simulink model "task3_lab7"  (R2024b)
settings: Solver=VariableStepAuto  StartTime=0.0  StopTime=10.0  RelTol=1e-3
settings Model: Creator=Beanie  LastModifiedBy=Beanie

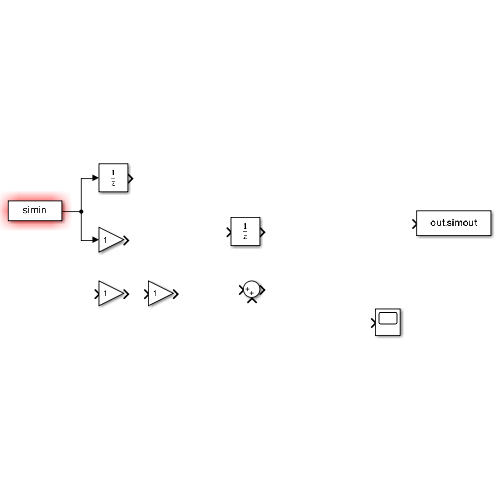
[thumbnail: Simulink's stored preview of the top-level diagram]
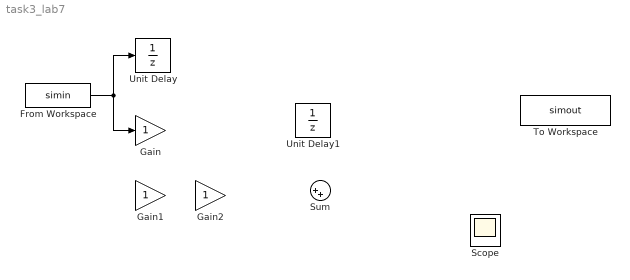
== system task3_lab7 ==
  From Workspace : FromWorkspace  VariableName=simin
  Gain : Gain
  Gain1 : Gain
  Gain2 : Gain
  Scope : Scope
  Sum : Sum  Inputs=|++
  To Workspace : ToWorkspace  VariableName=simout  SaveFormat=Timeseries  SampleTime=-1
  Unit Delay : UnitDelay  SampleTime=-1  HasFrameUpgradeWarning=on
  Unit Delay1 : UnitDelay  SampleTime=-1  HasFrameUpgradeWarning=on
  wires:
  From Workspace/1 -> Gain/1, Unit Delay/1
